simulink model "Grid_Subsystem"  (R2024b)
settings: Solver=VariableStepAuto  StartTime=0.0  StopTime=0.2  RelTol=1e-3
libraries: spsCurrentMeasurementLib x3, slpidlib x3, spsThreePhaseSeriesRLCBranchLib x2, spsGroundLib x2, spsabctodq0Lib x2, spsParallelRLCBranchLib x1, spsPLL3phLib x1, spsPWMGenerator2LevelLib x1, spsThreePhaseParallelRLCLoadLib x1, spsThreePhaseProgrammableVoltageSourceLib x1, spsThreePhaseVIMeasurementLib x1, spsUniversalBridgeLib x1
settings Model: Creator=Raju  LastModifiedBy=Raju

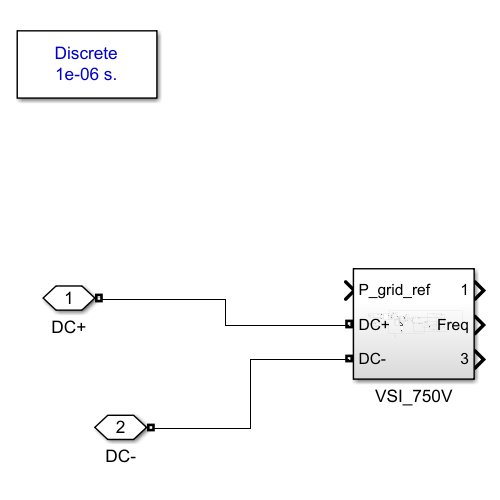
[thumbnail: Simulink's stored preview of the top-level diagram]
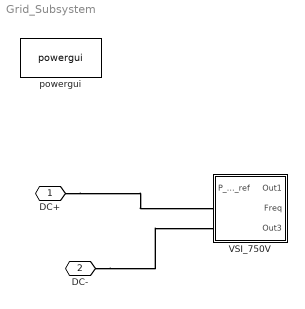
== system Grid_Subsystem ==
  VSI_750V : Subsystem
  powergui : spspowerguiLib/powergui  Priority=1  SimulationMode=Discrete  SampleTime=1e-6  frequency=60  Iterations=50  frequencyindice=50  Pbase=100e6  ErrMax=1e-4  UnitsV=kV  UnitsW=MW  buscounter=0  FunctionMessages=off  echomessages=off  EnableUseOfTLC=off  CurrentSourceSwitches=off  DisableSnubberDevices=off  DisableRonSwitches=off  DisableVfSwitches=off  DisplayEquations=off  AutomaticDiscreteSolvers=off  SolverType=Tustin/Backward Euler (TBE)  Interpol=off  ExternalGateDelay=off  methode=off  Ts=100  x0status=blocks  SPID=on  SwTol=0  HookPort=off  NonlinearTolerance=1e-4  nMaxIteration=100  ContinueOnMaxIteration=off  RestoreLinks=warning  ResistiveCurrentMeasurement=off  Frange=[0:2:500]  Ylog=off  Xlog=on  ShowGrid=off  save=off  variable=ZData  structure=0  ZoomFFT=off  StartTime=0.0  cycles=1  DisplayStyle=1  fundamental=60  FreqAxis=off  MaxFrequency=1000  frequencyindicesteady=1  RmsSteady=1  display=off
  DC+ : PMIOPort  Side=Left
  DC- : PMIOPort  Port=2  Side=Left
  connections:
  DC+/RConn1 -- VSI_750V/LConn1
  DC-/RConn1 -- VSI_750V/LConn2

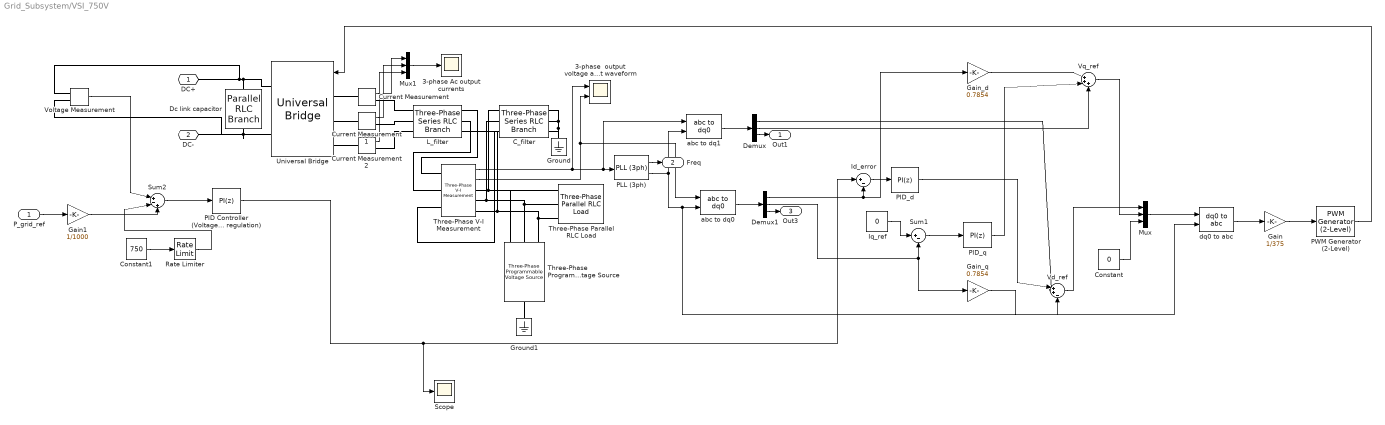
== system Grid_Subsystem/VSI_750V ==
  P_grid_ref : Inport
  3-phase  output voltage and current waveform : Scope  NumInputPorts=2
  3-phase Ac output currents : Scope
  C_filter : spsThreePhaseSeriesRLCBranchLib/Three-Phase Series RLC Branch  LConnTagsString=A|B|C  RConnTagsString=A|B|C  BranchType=RC  Resistance=1.5  Inductance=2.5e-3  Capacitance=25e-6  Measurements=None
  Constant : Constant  Value=0
  Constant1 : Constant  Value=750
  Current Measurement : spsCurrentMeasurementLib/Current Measurement  PhasorSimulation=off  OutputType=Complex  PSBequivalent=0
  Current Measurement1 : spsCurrentMeasurementLib/Current Measurement  PhasorSimulation=off  OutputType=Complex  PSBequivalent=0
  Current Measurement2 : spsCurrentMeasurementLib/Current Measurement  PhasorSimulation=off  OutputType=Complex  PSBequivalent=0
  Dc link capacitor : spsParallelRLCBranchLib/Parallel RLC Branch  LConnTagsString=a  RConnTagsString=__new0  BranchType=C  Resistance=1  Inductance=1e-3  SetiL0=off  InitialCurrent=0  Capacitance=2200e-6  Setx0=off  InitialVoltage=0  Measurements=None
  Demux : Demux  Outputs=3
  Demux1 : Demux  Outputs=3
  Gain : Gain  Gain=1/375
  Gain1 : Gain  Gain=1/1000
  Gain_d : Gain  Gain=0.7854
  Gain_q : Gain  Gain=0.7854
  Ground : spsGroundLib/Ground  LConnTagsString=a
  Ground1 : spsGroundLib/Ground  LConnTagsString=a
  Id_error : Sum  Inputs=|+-
  Iq_ref : Constant  Value=0
  L_filter : spsThreePhaseSeriesRLCBranchLib/Three-Phase Series RLC Branch  LConnTagsString=A|B|C  RConnTagsString=A|B|C  BranchType=RL  Resistance=0.05  Inductance=2.5e-3  Capacitance=1e-6  Measurements=None
  Mux : Mux  Inputs=3
  Mux1 : Mux  Inputs=3
  PID Controller (Voltage regulation) : slpidlib/PID Controller  Controller=PI  Form=Parallel  TimeDomain=Discrete-time  UseExternalTs=off  SampleTime=1e-6  IntegratorMethod=Forward Euler  FilterMethod=Forward Euler  ControllerParametersSource=internal  P=0.5  I=25  UseKiTs=off  D=0  UseExternalDerivativeSource=off  N=100  UseFilter=on  TunerSelectOption=Transfer Function Based (PID Tuner App)  InitialConditionSource=internal  InitialConditionForIntegrator=0  InitialConditionForFilter=0  DifferentiatorICPrevScaledInput=0  ExternalReset=none  TrackingMode=off  Kt=1  LimitOutput=on  SatLimitsSource=internal  UpperSaturationLimit=500  LowerSaturationLimit=0  LinearizeAsGain=on  AntiWindupMode=back-calculation  Kb=1  LimitIntegrator=off  UpperIntegratorSaturationLimit=inf  LowerIntegratorSaturationLimit=-inf  POutMin=[]  POutMax=[]  IOutMin=[]  IOutMax=[]  DOutMin=[]  DOutMax=[]  NOutMin=[]  NOutMax=[]  SumOutMin=[]  SumOutMax=[]  SaturationOutMin=[]  SaturationOutMax=[]  PParamMin=[]  PParamMax=[]  IParamMin=[]  IParamMax=[]  DParamMin=[]  DParamMax=[]  NParamMin=[]  NParamMax=[]  KbParamMin=[]  KbParamMax=[]  KtParamMin=[]  KtParamMax=[]  KbOutMin=[]  KbOutMax=[]  KtOutMin=[]  KtOutMax=[]  IntegratorOutMin=[]  IntegratorOutMax=[]  FilterOutMin=[]  FilterOutMax=[]  SumI1OutMin=[]  SumI1OutMax=[]  SumI2OutMin=[]  SumI2OutMax=[]  SumI3OutMin=[]  SumI3OutMax=[]  SumI4OutMin=[]  SumI4OutMax=[]  SumDOutMin=[]  SumDOutMax=[]  DifferentiatorOutMin=[]  DifferentiatorOutMax=[]  FilterDiffOutCoefMin=[]  FilterDiffOutCoefMax=[]  ReciprocalOutMin=[]  ReciprocalOutMax=[]  SumDenOutMin=[]  SumDenOutMax=[]  SumNumOutMin=[]  SumNumOutMax=[]  DivideOutMin=[]  DivideOutMax=[]  UdiffTsProdOutMin=[]  UdiffTsProdOutMax=[]  NTsProdOutMin=[]  NTsProdOutMax=[]  UintegralTsProdOutMin=[]  UintegralTsProdOutMax=[]  UngainTsProdOutMin=[]  UngainTsProdOutMax=[]  ClampingZeroOutDataTypeStr=Inherit: Inherit via back propagation  ClampingZeroOutMin=[]  ClampingZeroOutMax=[]  FilterDenConstantOutDataTypeStr=Inherit: Inherit via back propagation  FilterDenConstantOutMin=[]  FilterDenConstantOutMax=[]  PCopyOutDataTypeStr=Inherit: Inherit via back propagation  PCopyOutMin=[]  PCopyOutMax=[]  NCopyOutDataTypeStr=Inherit: Inherit via back propagation  NCopyOutMin=[]  NCopyOutMax=[]  IntegratorContinuousStateAttributes=''  IntegratorStateMustResolveToSignalObject=off  IntegratorRTWStateStorageClass=Auto  FilterContinuousStateAttributes=''  FilterStateMustResolveToSignalObject=off  FilterRTWStateStorageClass=Auto  ParallelPVariant=InternalParameters  IdealPVariant=Disabled  IVariant=InternalParameters  DVariant=Disabled  IntegratorVariant=Discrete  SatVariant=Enabled  AWVariant=BackCalculation  PCopyVariant=Disabled  TRVariant=Disabled  FdbkBlocksVariant=Forward  IdealPFdbkVariant=Disabled  SatFdbkVariant=Disabled  DerivativeFilterVariant=Disabled  NVariant=Disabled  NCopyVariant=Disabled_SignalSpec  FilterICVariant=Disabled  IntegratorICVariant=InternalICs  ExternalResetVariant=Disabled  TRSumVariant=Passthrough  SumFdbkVariant=Disabled  SumVariant=Sum_PI  TsampFilterVariant=InternalTs  TsampNgainVariant=Passthrough  TsampIntegralVariant=Disabled_SignalSpec  ExternalSaturationOutDataTypeStr=Inherit: Same as second input  DerivativeSourceVariant=Disabled  PreIntVariant=InternalPreInt
  PID_d : slpidlib/PID Controller  Controller=PI  Form=Parallel  TimeDomain=Discrete-time  UseExternalTs=off  SampleTime=1e-6  IntegratorMethod=Forward Euler  FilterMethod=Forward Euler  ControllerParametersSource=internal  P=5  I=100  UseKiTs=off  D=0  UseExternalDerivativeSource=off  N=100  UseFilter=on  TunerSelectOption=Transfer Function Based (PID Tuner App)  InitialConditionSource=internal  InitialConditionForIntegrator=0  InitialConditionForFilter=0  DifferentiatorICPrevScaledInput=0  ExternalReset=none  TrackingMode=off  Kt=1  LimitOutput=on  SatLimitsSource=internal  UpperSaturationLimit=500  LowerSaturationLimit=-500  LinearizeAsGain=on  AntiWindupMode=none  Kb=1  LimitIntegrator=off  UpperIntegratorSaturationLimit=inf  LowerIntegratorSaturationLimit=-inf  POutMin=[]  POutMax=[]  IOutMin=[]  IOutMax=[]  DOutMin=[]  DOutMax=[]  NOutMin=[]  NOutMax=[]  SumOutMin=[]  SumOutMax=[]  SaturationOutMin=[]  SaturationOutMax=[]  PParamMin=[]  PParamMax=[]  IParamMin=[]  IParamMax=[]  DParamMin=[]  DParamMax=[]  NParamMin=[]  NParamMax=[]  KbParamMin=[]  KbParamMax=[]  KtParamMin=[]  KtParamMax=[]  KbOutMin=[]  KbOutMax=[]  KtOutMin=[]  KtOutMax=[]  IntegratorOutMin=[]  IntegratorOutMax=[]  FilterOutMin=[]  FilterOutMax=[]  SumI1OutMin=[]  SumI1OutMax=[]  SumI2OutMin=[]  SumI2OutMax=[]  SumI3OutMin=[]  SumI3OutMax=[]  SumI4OutMin=[]  SumI4OutMax=[]  SumDOutMin=[]  SumDOutMax=[]  DifferentiatorOutMin=[]  DifferentiatorOutMax=[]  FilterDiffOutCoefMin=[]  FilterDiffOutCoefMax=[]  ReciprocalOutMin=[]  ReciprocalOutMax=[]  SumDenOutMin=[]  SumDenOutMax=[]  SumNumOutMin=[]  SumNumOutMax=[]  DivideOutMin=[]  DivideOutMax=[]  UdiffTsProdOutMin=[]  UdiffTsProdOutMax=[]  NTsProdOutMin=[]  NTsProdOutMax=[]  UintegralTsProdOutMin=[]  UintegralTsProdOutMax=[]  UngainTsProdOutMin=[]  UngainTsProdOutMax=[]  ClampingZeroOutDataTypeStr=Inherit: Inherit via back propagation  ClampingZeroOutMin=[]  ClampingZeroOutMax=[]  FilterDenConstantOutDataTypeStr=Inherit: Inherit via back propagation  FilterDenConstantOutMin=[]  FilterDenConstantOutMax=[]  PCopyOutDataTypeStr=Inherit: Inherit via back propagation  PCopyOutMin=[]  PCopyOutMax=[]  NCopyOutDataTypeStr=Inherit: Inherit via back propagation  NCopyOutMin=[]  NCopyOutMax=[]  IntegratorContinuousStateAttributes=''  IntegratorStateMustResolveToSignalObject=off  IntegratorRTWStateStorageClass=Auto  FilterContinuousStateAttributes=''  FilterStateMustResolveToSignalObject=off  FilterRTWStateStorageClass=Auto  ParallelPVariant=InternalParameters  IdealPVariant=Disabled  IVariant=InternalParameters  DVariant=Disabled  IntegratorVariant=Discrete  SatVariant=Enabled  AWVariant=Passthrough  PCopyVariant=Disabled  TRVariant=Disabled  FdbkBlocksVariant=Forward  IdealPFdbkVariant=Disabled  SatFdbkVariant=Disabled  DerivativeFilterVariant=Disabled  NVariant=Disabled  NCopyVariant=Disabled_SignalSpec  FilterICVariant=Disabled  IntegratorICVariant=InternalICs  ExternalResetVariant=Disabled  TRSumVariant=Passthrough  SumFdbkVariant=Disabled  SumVariant=Sum_PI  TsampFilterVariant=InternalTs  TsampNgainVariant=Passthrough  TsampIntegralVariant=Disabled_SignalSpec  ExternalSaturationOutDataTypeStr=Inherit: Same as second input  DerivativeSourceVariant=Disabled  PreIntVariant=InternalPreInt
  PID_q : slpidlib/PID Controller  Controller=PI  Form=Parallel  TimeDomain=Discrete-time  UseExternalTs=off  SampleTime=1e-6  IntegratorMethod=Forward Euler  FilterMethod=Forward Euler  ControllerParametersSource=internal  P=5  I=100  UseKiTs=off  D=0  UseExternalDerivativeSource=off  N=100  UseFilter=on  TunerSelectOption=Transfer Function Based (PID Tuner App)  InitialConditionSource=internal  InitialConditionForIntegrator=0  InitialConditionForFilter=0  DifferentiatorICPrevScaledInput=0  ExternalReset=none  TrackingMode=off  Kt=1  LimitOutput=on  SatLimitsSource=internal  UpperSaturationLimit=500  LowerSaturationLimit=-500  LinearizeAsGain=on  AntiWindupMode=none  Kb=1  LimitIntegrator=off  UpperIntegratorSaturationLimit=inf  LowerIntegratorSaturationLimit=-inf  POutMin=[]  POutMax=[]  IOutMin=[]  IOutMax=[]  DOutMin=[]  DOutMax=[]  NOutMin=[]  NOutMax=[]  SumOutMin=[]  SumOutMax=[]  SaturationOutMin=[]  SaturationOutMax=[]  PParamMin=[]  PParamMax=[]  IParamMin=[]  IParamMax=[]  DParamMin=[]  DParamMax=[]  NParamMin=[]  NParamMax=[]  KbParamMin=[]  KbParamMax=[]  KtParamMin=[]  KtParamMax=[]  KbOutMin=[]  KbOutMax=[]  KtOutMin=[]  KtOutMax=[]  IntegratorOutMin=[]  IntegratorOutMax=[]  FilterOutMin=[]  FilterOutMax=[]  SumI1OutMin=[]  SumI1OutMax=[]  SumI2OutMin=[]  SumI2OutMax=[]  SumI3OutMin=[]  SumI3OutMax=[]  SumI4OutMin=[]  SumI4OutMax=[]  SumDOutMin=[]  SumDOutMax=[]  DifferentiatorOutMin=[]  DifferentiatorOutMax=[]  FilterDiffOutCoefMin=[]  FilterDiffOutCoefMax=[]  ReciprocalOutMin=[]  ReciprocalOutMax=[]  SumDenOutMin=[]  SumDenOutMax=[]  SumNumOutMin=[]  SumNumOutMax=[]  DivideOutMin=[]  DivideOutMax=[]  UdiffTsProdOutMin=[]  UdiffTsProdOutMax=[]  NTsProdOutMin=[]  NTsProdOutMax=[]  UintegralTsProdOutMin=[]  UintegralTsProdOutMax=[]  UngainTsProdOutMin=[]  UngainTsProdOutMax=[]  ClampingZeroOutDataTypeStr=Inherit: Inherit via back propagation  ClampingZeroOutMin=[]  ClampingZeroOutMax=[]  FilterDenConstantOutDataTypeStr=Inherit: Inherit via back propagation  FilterDenConstantOutMin=[]  FilterDenConstantOutMax=[]  PCopyOutDataTypeStr=Inherit: Inherit via back propagation  PCopyOutMin=[]  PCopyOutMax=[]  NCopyOutDataTypeStr=Inherit: Inherit via back propagation  NCopyOutMin=[]  NCopyOutMax=[]  IntegratorContinuousStateAttributes=''  IntegratorStateMustResolveToSignalObject=off  IntegratorRTWStateStorageClass=Auto  FilterContinuousStateAttributes=''  FilterStateMustResolveToSignalObject=off  FilterRTWStateStorageClass=Auto  ParallelPVariant=InternalParameters  IdealPVariant=Disabled  IVariant=InternalParameters  DVariant=Disabled  IntegratorVariant=Discrete  SatVariant=Enabled  AWVariant=Passthrough  PCopyVariant=Disabled  TRVariant=Disabled  FdbkBlocksVariant=Forward  IdealPFdbkVariant=Disabled  SatFdbkVariant=Disabled  DerivativeFilterVariant=Disabled  NVariant=Disabled  NCopyVariant=Disabled_SignalSpec  FilterICVariant=Disabled  IntegratorICVariant=InternalICs  ExternalResetVariant=Disabled  TRSumVariant=Passthrough  SumFdbkVariant=Disabled  SumVariant=Sum_PI  TsampFilterVariant=InternalTs  TsampNgainVariant=Passthrough  TsampIntegralVariant=Disabled_SignalSpec  ExternalSaturationOutDataTypeStr=Inherit: Same as second input  DerivativeSourceVariant=Disabled  PreIntVariant=InternalPreInt
  PLL (3ph) : spsPLL3phLib/PLL (3ph)  Fmin=45  Par_Init=[0, 50]  ParK=[180, 3200, 1]  TcD=1e-4  MaxRateChangeFreq=12  FilterCutOffFreq=25  Ts=1e-4  AGC=on
  PWM Generator (2-Level) : spsPWMGenerator2LevelLib/PWM Generator (2-Level)  ModulatorType=Three-phase bridge (6 pulses)  ModulatorMode=Unsynchronized  Fc=10000  Pc=90  nF=27  MinMax="[ -1  1 ]"  SamplingTechnique=Natural  ModulatingSignals=off  m=0.8  Freq=60  Phase=0  Ts=0  ShowCarrierOutport=off
  Rate Limiter : RateLimiter  RisingSlewLimit=75000  FallingSlewLimit=-75000  SampleTimeMode=inherited  InitialCondition=750
  Scope : Scope
  Sum1 : Sum  Inputs=|+-
  Sum2 : Sum  Inputs=|+-+
  Three-Phase Parallel RLC Load : spsThreePhaseParallelRLCLoadLib/Three-Phase Parallel RLC Load  LConnTagsString=A|B|C  Configuration=Y (grounded)  NominalVoltage=400  Vabc=[1e3 1e3 1e3]  Vabcp=[1e3 1e3 1e3]  NominalFrequency=50  UnbalancedPower=off  ActivePower=20000  InductivePower=0  CapacitivePower=0  Pabc=[10e3 9e3 11e3]  QLabc=[100 90 110]  QCabc=[100 90 110]  Pabcp=[10e3 9e3 11e3]  QLabcp=[100 90 110]  QCabcp=[100 90 110]  Measurements=None  LoadType=constant Z
  Three-Phase Programmable Voltage Source : spsThreePhaseProgrammableVoltageSourceLib/Three-Phase Programmable Voltage Source  PositiveSequence="[400  0 50]"  VariationEntity=None  VariationType=Table of time-amplitude pairs  VariationTypeAlt=Step  VariationStep=0.5  VariationRate=10  VariationMagnitude=0.3  VariationFrequency=2  VariationTiming=[1 2]  VariationPhaseA=off  Amplitudes=[1 0.8 1.2 1.0]  TimeValues=[0 0.1 0.15 0.2]  HarmonicGeneration=off  HarmonicA=[3 0.2 -25 0]  HarmonicB=[2 0.15 35 2]  Timing="[0.05  3]"  BusType=swing  Pref=0  Qref=0  Qmin=-inf  Qmax=inf
  Three-Phase V-I Measurement : spsThreePhaseVIMeasurementLib/Three-Phase V-I Measurement  VoltageMeasurement=phase-to-ground  SetLabelV=off  LabelV=Vabc  Vpu=off  VpuLL=off  CurrentMeasurement=yes  SetLabelI=off  LabelI=Iabc  Ipu=off  Pbase=100e6  Vbase=500e3  OutputType=Complex  PhasorSimulation=off  PSBequivalent=0
  Universal Bridge : spsUniversalBridgeLib/Universal Bridge  Arms=3  SnubberResistance=1e5  SnubberCapacitance=inf  Device=IGBT / Diodes  Ron=1e-3  Lon=0  ForwardVoltages="[  0  0  ]"  ForwardVoltage=0  GTOparameters=[ 10e-6 , 20e-6 ]  IGBTparameters=[ 1e-6 , 2e-6 ]  Measurements=None  Measurements_2=None  converterType=Rectifier
  Vd_ref : Sum  Inputs=|++-
  Voltage Measurement : spsVoltageMeasurementLib/Voltage Measurement  PhasorSimulation=off  OutputType=Complex  PSBequivalent=0
  Vq_ref : Sum  Inputs=|+++
  abc to dq0 : spsabctodq0Lib/abc to dq0  Alignment=Aligned with phase A axis
  abc to dq1 : spsabctodq0Lib/abc to dq0  Alignment=Aligned with phase A axis
  dq0 to abc : spsdq0toabcLib/dq0 to abc  Alignment=Aligned with phase A axis
  DC+ : PMIOPort  Side=Left
  DC- : PMIOPort  Port=2  Side=Left
  Out1 : Outport
  Freq : Outport  Port=2
  Out3 : Outport  Port=3
  wires:
  Gain1/1 -> Sum2/3
  Voltage Measurement/1 -> Sum2/1
  Mux/1 -> dq0 to abc/1
  Vd_ref/1 -> Mux/1
  Rate Limiter/1 -> Sum2/2
  Mux1/1 -> 3-phase Ac output currents/1
  PID_d/1 -> Vd_ref/1
  PWM Generator (2-Level)/1 -> Universal Bridge/1
  Sum2/1 -> PID Controller (Voltage regulation)/1
  PID Controller (Voltage regulation)/1 -> Scope/1, Id_error/1
  PLL (3ph)/2 -> dq0 to abc/2, abc to dq0/2, abc to dq1/2
  Demux/1 -> Vd_ref/2
  Constant1/1 -> Rate Limiter/1
  Demux1/1 -> Gain_d/1, Id_error/2
  Current Measurement/1 -> Mux1/1
  Sum1/1 -> PID_q/1
  Current Measurement2/1 -> Mux1/3
  PLL (3ph)/1 -> Freq/1
  Gain_d/1 -> Vq_ref/1
  PID_q/1 -> Vq_ref/2
  Demux/3 -> Out1/1
  Three-Phase V-I Measurement/1 -> 3-phase  output voltage and current waveform/1, abc to dq1/1, PLL (3ph)/1
  Gain_q/1 -> Vd_ref/3
  Iq_ref/1 -> Sum1/1
  Demux1/2 -> Gain_q/1, Sum1/2
  Demux/2 -> Vq_ref/3
  Constant/1 -> Mux/3
  Vq_ref/1 -> Mux/2
  dq0 to abc/1 -> Gain/1
  Current Measurement1/1 -> Mux1/2
  abc to dq1/1 -> Demux/1
  Gain/1 -> PWM Generator (2-Level)/1
  Id_error/1 -> PID_d/1
  Demux1/3 -> Out3/1
  abc to dq0/1 -> Demux1/1
  Three-Phase V-I Measurement/2 -> 3-phase  output voltage and current waveform/2, abc to dq0/1
  P_grid_ref/1 -> Gain1/1
  connections:
  Dc link capacitor/RConn1 -- DC-/RConn1 -- Voltage Measurement/LConn2 -- Universal Bridge/RConn2
  Voltage Measurement/LConn1 -- DC+/RConn1 -- Universal Bridge/RConn1 -- Dc link capacitor/LConn1
  Three-Phase V-I Measurement/RConn2 -- C_filter/LConn2 -- Three-Phase Programmable Voltage Source/RConn2 -- Three-Phase Parallel RLC Load/LConn2
  C_filter/LConn1 -- Three-Phase V-I Measurement/RConn1 -- Three-Phase Programmable Voltage Source/RConn1 -- Three-Phase Parallel RLC Load/LConn1
  C_filter/LConn3 -- Three-Phase V-I Measurement/RConn3 -- Three-Phase Programmable Voltage Source/RConn3 -- Three-Phase Parallel RLC Load/LConn3
  C_filter/RConn3 -- C_filter/RConn1 -- C_filter/RConn2 -- Ground/LConn1
  Ground1/LConn1 -- Three-Phase Programmable Voltage Source/LConn1
  Universal Bridge/LConn3 -- Current Measurement2/LConn1
  L_filter/LConn1 -- Current Measurement/RConn1
  Current Measurement1/LConn1 -- Universal Bridge/LConn2
  Three-Phase V-I Measurement/LConn1 -- L_filter/RConn1
  Current Measurement2/RConn1 -- L_filter/LConn3
  Current Measurement/LConn1 -- Universal Bridge/LConn1
  Three-Phase V-I Measurement/LConn3 -- L_filter/RConn3
  Three-Phase V-I Measurement/LConn2 -- L_filter/RConn2
  Current Measurement1/RConn1 -- L_filter/LConn2
